simulink model "PandaRL"  (R2025b)
settings: Solver=FixedStepDiscrete  StartTime=0.0  StopTime=20  FixedStep=0.05  RelTol=1e-3
model workspace (MAT data in the model file):
  pandaTemplate : object (value not decoded)
undefined symbols (not defined in the file or in its folder): episodeInitialObservation, episodeInitialState
libraries: rllib x1
settings Model: Creator=Compu  LastModifiedBy=Compu

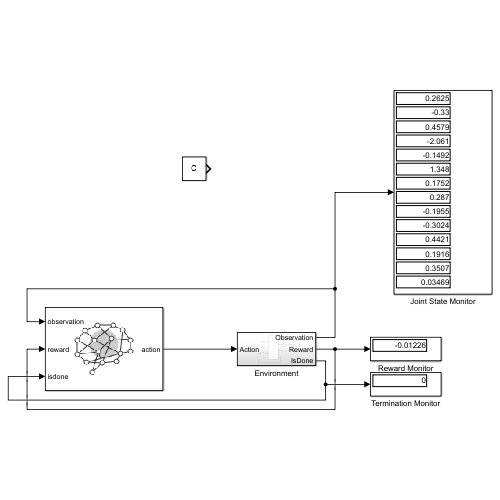
[thumbnail: Simulink's stored preview of the top-level diagram]
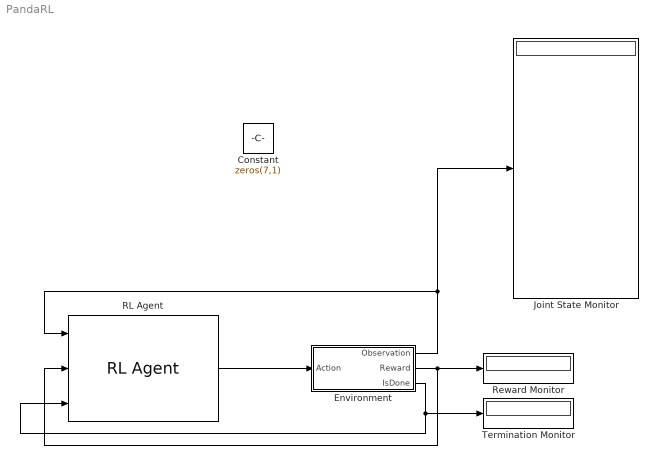
== system PandaRL ==
  Constant : Constant  Value=zeros(7,1)
  Environment : Subsystem
  Joint State Monitor : Display
  RL Agent : rllib/RL Agent  Agent=agentObj  ExternalActionAsInput=off  ProvideLastAction=off  ProvideCumRwd=off  TreatAsDirectFeedthrough=on  UseStrictObservationDataTypes=off
  Reward Monitor : Display
  Termination Monitor : Display
  wires:
  Environment/1(Observation) -> Joint State Monitor/1, RL Agent/1
  Environment/2(Reward) -> Reward Monitor/1, RL Agent/2
  Environment/3(IsDone) -> Termination Monitor/1, RL Agent/3
  RL Agent/1 -> Environment/1(Action)

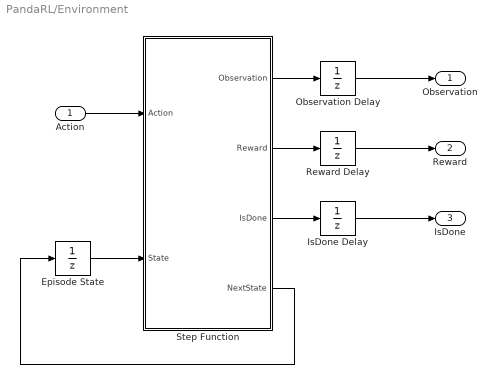
== system PandaRL/Environment ==
  Action : Inport  PortDimensions=[7 1]
  Episode State : UnitDelay  InitialCondition=episodeInitialState  SampleTime=0.05  HasFrameUpgradeWarning=on
  IsDone Delay : UnitDelay  InitialCondition=false  SampleTime=0.05  HasFrameUpgradeWarning=on
  Observation Delay : UnitDelay  InitialCondition=episodeInitialObservation  SampleTime=0.05  HasFrameUpgradeWarning=on
  Reward Delay : UnitDelay  SampleTime=0.05  HasFrameUpgradeWarning=on
  Step Function : MATLAB Function  TreatAsAtomicUnit=on
  Observation : Outport
  Reward : Outport  Port=2
  IsDone : Outport  Port=3
  wires:
  Action/1 -> Step Function/1(Action)
  Episode State/1 -> Step Function/2(State)
  Step Function/1(Observation) -> Observation Delay/1
  Step Function/2(Reward) -> Reward Delay/1
  Step Function/3(IsDone) -> IsDone Delay/1
  Step Function/4(NextState) -> Episode State/1
  Observation Delay/1 -> Observation/1
  Reward Delay/1 -> Reward/1
  IsDone Delay/1 -> IsDone/1

== matlab function PandaRL/Environment/Step Function ==
  data: Action input; Observation output; State input; Reward output; IsDone output; NextState output

function [Observation, Reward, IsDone, NextState] = fcn(Action, State)
% Panda RL environment interface.
% Reuses the existing environment implementation.

coder.extrinsic('environment.simulinkStep');

Observation = zeros(14,1);
Reward = 0;
IsDone = false;
NextState = zeros(19,1);

[Observation, Reward, IsDone, NextState] = ...
    environment.simulinkStep(Action, State);

end
